simulink model "tema3_reglare"  (R2026a)
settings: Solver=ode45  StopTime=0.12  MaxStep=1e-5
values from neighbouring files (symbols this model uses):
  freq = 800    [tema3.m]
  u_out = 20    [proiect.m]    (also in tema2_simscape.m; tema3.m)
undefined symbols (not defined in the file or in its folder): den, den_c, num, num_c
settings Model: Creator=Fer Alexandru  LastModifiedBy=Fer Alexandru

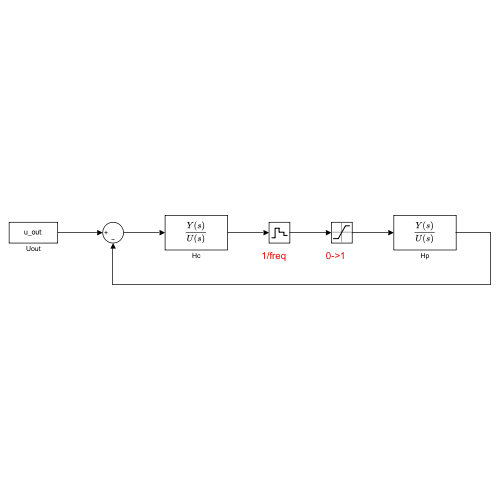
[thumbnail: Simulink's stored preview of the top-level diagram]
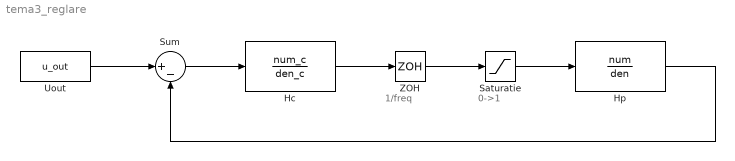
== system tema3_reglare ==
  note: 1/freq
  note: 0->1
  Hc : TransferFcn  Numerator=num_c  Denominator=den_c
  Hp : TransferFcn  Numerator=num  Denominator=den
  Saturatie : Saturate  UpperLimit=1  LowerLimit=0
  Sum : Sum  Inputs=|+-
  Uout : Constant  Value=u_out
  ZOH : ZeroOrderHold  SampleTime=1/freq
  wires:
  Uout/1 -> Sum/1
  Sum/1 -> Hc/1
  Hc/1 -> ZOH/1
  ZOH/1 -> Saturatie/1
  Saturatie/1 -> Hp/1
  Hp/1 -> Sum/2
